simulink model "autopilot_closed_loop"  (R2024a)
settings: Solver=VariableStepAuto  StartTime=0.0  StopTime=1000  RelTol=1e-3
values from neighbouring files (symbols this model uses):
  A = [-0.0156 0.0101 0 -9.81; -0.1367 -1.9635 186 0; 0.000948 -0.02555 -3.6668 0;0 0 1 0]    [longitudinal_pole_placement.m]
  B = [0; 0.1351; -0.14456; 0]    [longitudinal_pole_placement.m]
  C = [1 0 0 0; 0 1 0 0; 0 0 1 0; 0 0 0 1]    [longitudinal_pole_placement.m]
  D = [0; 0; 0; 0]    [longitudinal_pole_placement.m]
  K = place(A, B, poles_desires)    [longitudinal_pole_placement.m]
settings Model: Creator=yanis  LastModifiedBy=yanis

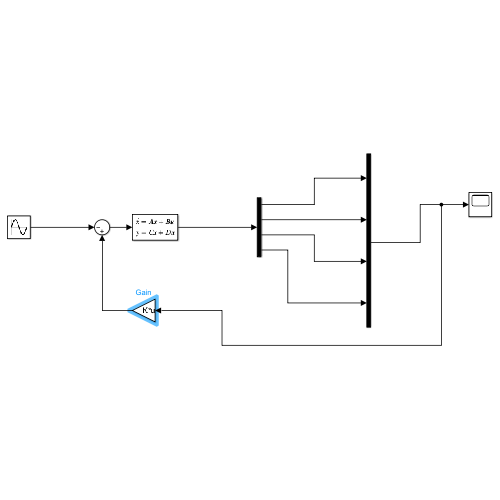
[thumbnail: Simulink's stored preview of the top-level diagram]
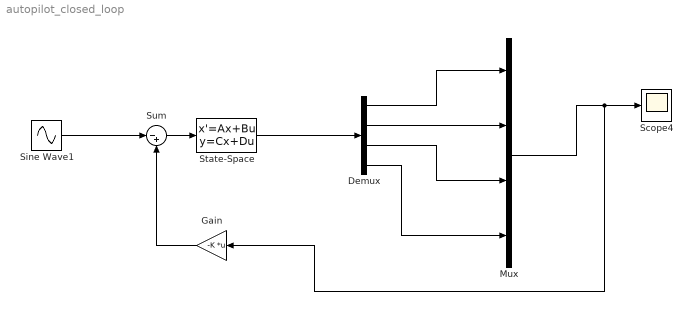
== system autopilot_closed_loop ==
  Demux : Demux
  Gain : Gain  Gain=-K  Multiplication=Matrix(K*u)
  Mux : Mux
  Scope4 : Scope
  Sine Wave1 : Sin  Amplitude=0.1  Frequency=0.099  SampleTime=0
  State-Space : StateSpace  A=A  B=B  C=C  D=D  InitialCondition=[0.1,0,0,0.01]
  Sum : Sum  Inputs=|-+
  wires:
  State-Space/1 -> Demux/1
  Demux/3 -> Mux/3
  Demux/1 -> Mux/1
  Mux/1 -> Gain/1, Scope4/1
  Demux/4 -> Mux/4
  Demux/2 -> Mux/2
  Sum/1 -> State-Space/1
  Sine Wave1/1 -> Sum/1
  Gain/1 -> Sum/2
